simulink model "Elevator_simulation_regenerative_braking_completed"  (R2025b)
settings: Solver=VariableStepAuto  StartTime=0.0  StopTime=41  RelTol=1e-3
model workspace (MAT data in the model file):
  AFE_id_ref_profile = timeseries
  AFE_id_ref_profile.Name = 'unnamed'
  AFE_id_ref_profile.DataInfo = tsdata.datametadata
  AFE_id_ref_profile.DataInfo.Interpolation = tsdata.interpolation
  AFE_id_ref_profile.DataInfo.Interpolation.Fhandle : function handle (value not decoded)
  AFE_id_ref_profile.DataInfo.Interpolation.Name = 'linear'
  AFE_id_ref_profile.TimeInfo = tsdata.timemetadata
  AFE_id_ref_profile.TimeInfo.Length = 6
  AFE_id_ref_profile.TimeInfo.DuplicateTimes = 0
  AFE_id_ref_profile.TimeInfo.Time_ = [0; 0.1; 2; 3; 3.1; 5]
  AFE_id_ref_profile.TimeInfo.Initialized = 1
  AFE_id_ref_profile.QualityInfo = tsdata.qualmetadata
  AFE_id_ref_profile.Data_ = [0.5; 0.5; 0.5; 0.5; -0.5; -0.5]
  G = 10
  Jeq = 0.8325
  Tgravity = 27.25
  eta = 0.9
  g = 9.81
  mc = 500
  mcw = 600
  mp = 200
  r = 0.25
  regen_enable = timeseries
  regen_enable.Name = 'Regenerative braking enable'
  regen_enable.DataInfo = tsdata.datametadata
  regen_enable.DataInfo.Interpolation = tsdata.interpolation
  regen_enable.DataInfo.Interpolation.Fhandle : function handle (value not decoded)
  regen_enable.DataInfo.Interpolation.Name = 'linear'
  regen_enable.TimeInfo = tsdata.timemetadata
  regen_enable.TimeInfo.Length = 4
  regen_enable.TimeInfo.DuplicateTimes = 0
  regen_enable.TimeInfo.Time_ = [0; 0.2; 2.5; 5]
  regen_enable.TimeInfo.Initialized = 1
  regen_enable.QualityInfo = tsdata.qualmetadata
  regen_enable.Data_ = reshape([0 0 1 1], [1 1 4])
  sc_Pdead = 50
  sc_Plimit = 100000
  sc_Vinit = 360
  sc_Vmax = 470
  sc_Vmin = 300
  sc_dV = 10
  sc_enable = 1
  sc_kdis = 0.5
  sc_tauP = 0.02
  sc_tauV = 0.001
  speed_cmd = timeseries
  speed_cmd.Name = 'Elevator speed reference (round trip)'
  speed_cmd.DataInfo = tsdata.datametadata
  speed_cmd.DataInfo.Interpolation = tsdata.interpolation
  speed_cmd.DataInfo.Interpolation.Fhandle : function handle (value not decoded)
  speed_cmd.DataInfo.Interpolation.Name = 'linear'
  speed_cmd.TimeInfo = tsdata.timemetadata
  speed_cmd.TimeInfo.Length = 9
  speed_cmd.TimeInfo.DuplicateTimes = 0
  speed_cmd.TimeInfo.Time_ = [0; 8.001; 10.001; 18.001; 22; 30.001; 32.001; 40.001; 41]
  speed_cmd.TimeInfo.Initialized = 1
  speed_cmd.QualityInfo = tsdata.qualmetadata
  speed_cmd.Data_ = [0; 764; 764; 0; 0; -764; -764; 0; 0]
  speed_mps = timeseries
  speed_mps.Name = 'unnamed'
  speed_mps.DataInfo = tsdata.datametadata
  speed_mps.DataInfo.Interpolation = tsdata.interpolation
  speed_mps.DataInfo.Interpolation.Fhandle : function handle (value not decoded)
  speed_mps.DataInfo.Interpolation.Name = 'linear'
  speed_mps.TimeInfo = tsdata.timemetadata
  speed_mps.TimeInfo.Length = 4
  speed_mps.TimeInfo.DuplicateTimes = 0
  speed_mps.TimeInfo.Time_ = [0; 0.2; 2.5; 5]
  speed_mps.TimeInfo.Initialized = 1
  speed_mps.QualityInfo = tsdata.qualmetadata
  speed_mps.Data_ = [0; 2; 2; 0]
libraries: slpidlib x3, spsThreePhaseSeriesRLCBranchLib x3, spsThreePhaseVIMeasurementLib x3, spsControlledCurrentSourceLib x2, spsUniversalBridgeLib x2, spsVoltageMeasurementLib x2, autolibdcdc x1, spsCurrentMeasurementLib x1, eeGeneralControl x1, spsPLL3phLib x1, eePmsmFieldOrientedControl x1, spsPWMGenerator2LevelLib x1
settings Model: SimulationMode=rapid-accelerator  Creator=kesav  LastModifiedBy=kesava-d-raj
settings SolverCC: ZeroCrossAlgorithm=Adaptive

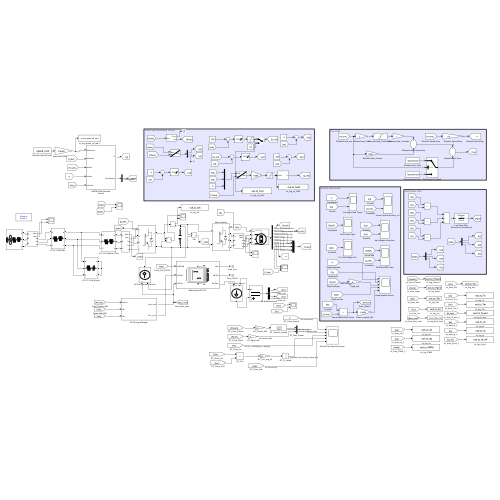
[thumbnail: Simulink's stored preview of the top-level diagram]
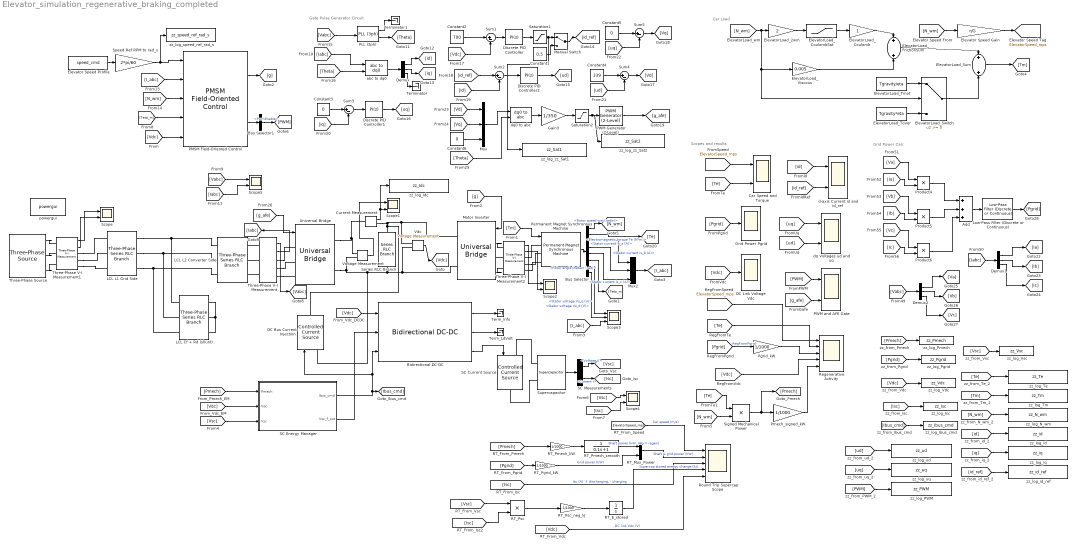
== system Elevator_simulation_regenerative_braking_completed ==
  note: Scopes and results
  note: Grid Power Calc
  note: Car Load
  note: Gate Pulse Generator Circuit
  Add : Sum  Inputs=+++
  Bidirectional DC-DC : autolibdcdc/Bidirectional DC-DC  Tc=1/1000  Vinit=0  Plimit=100000  param_loss=Single efficiency measurement  eff=98  v_loss_bp=[0 200 400 600 800 1000]  i_loss_bp=[0 25 50 75 100]  losses_table=[100 100 100 100 100;100 150 200 250 300;100 200 300 400 500;100 250 400 550 700;100 300 500 700 900;100 350 600 850 1100]  v_eff_bp=[200 400 600 800 1000]  i_eff_bp=[25 50 75 100]  efficiency_table=[96.2 98.1 98.7 99;98.1 99 99.4 99.5;98.7 99.4 99.6 99.7;99 99.5 99.7 99.8;99.2 99.6 99.7 99.8]  x_v_bp=[-1000 -800 -600 -400 -200 200 400 600 800 1000]  x_i_bp=[-100 -75 -50 -25 25 50 75 100]  x_losses_mat=[200.400801603196 225.67703109328 200.803212851408 201.612903225806 199.999999999997 200 225 200;160.320641282556 180.541624874624 201.005025125625 202.020202020203 200 200 180 160;180.541624874624 180.722891566267 181.086519114686 197.568389057748 194.999999999999 179.999999999997 180 180;201.005025125625 181.086519114686 202.020202020203 193.67991845056 190 200 179.999999999997 200;202.020202020203 197.568389057748 193.67991845056 197.505197505197 190 190 194.999999999999 200;200 194.999999999999 190 190 197.505197505197 193.67991845056 197.568389057748 202.020202020203;200 179.999999999997 200 190 193.67991845056 202.020202020203 181.086519114686 201.005025125625;180 180 179.999999999997 194.999999999999 197.568389057748 181.086519114686 180.722891566267 180.541624874624;160 180 200 200 202.020202020203 201.005025125625 180.541624874624 160.320641282556;200 225 200 199.999999999997 201.612903225806 200.803212851408 225.67703109328 200.400801603196]  RefBlkName='autolibdcdc/Bidirectional DC-DC'  CalLossMapData={'BaseCageProjectFileName','';'BaseMbcProjectFileName','';'TaskName','Calibrate Inverter Loss Map';'ChildTasks',{{'DataName','';'TaskName','Import Loss Data'},{'TaskName','Generate Response Models'},{'TaskName','Generate Calibration'},{'TaskName','Update Block Parameters'}}}
  Bus Selector : BusSelector  OutputSignals=Rotor speed wm (rad/s),Electromagnetic torque Te (N*m),Stator current is_a (A),Stator current is_b (A),Stator current is_c (A),Rotor angle thetam (rad),Stator voltage Vs_q (V),Stator voltage Vs_d (V)
  Bus Selector1 : BusSelector  OutputSignals=PwmEnable
  Car Speed and Torque : Scope  NumInputPorts=2
      settings: ActiveDisplayYMinimum=-2.5140849185806631  ActiveDisplayYMaximum=2.51411750297212
  Constant1 : Constant  Value=0.5
  Constant2 : Constant  Value=700
  Constant3 : Constant  Value=0
  Constant4 : Constant  Value=339
  Constant5 : Constant  Value=0
  Constant6 : Constant  Value=0
  Current Measurement : spsCurrentMeasurementLib/Current Measurement  PhasorSimulation=off  OutputType=Complex  PSBequivalent=0
  DC Bus Current Injection : spsControlledCurrentSourceLib/Controlled Current Source  Initialize=on  Source_Type=AC  Amplitude=0  Phase=0  Frequency=0  Measurements=None
  DC Link Voltage Vdc : Scope
      settings: ActiveDisplayYMinimum=572.34967767738488  ActiveDisplayYMaximum=718.84953066041635  DataLoggingVariableName=ScopeData2
  Demux : Demux  Outputs=3
  Demux1 : Demux  Outputs=3
  Demux2 : Demux  Outputs=3
  Discrete PID Controller : slpidlib/PID Controller  Controller=PI  Form=Parallel  TimeDomain=Discrete-time  UseExternalTs=off  SampleTime=1e-4  IntegratorMethod=Forward Euler  FilterMethod=Forward Euler  ControllerParametersSource=internal  P=0.5  I=15  UseKiTs=off  D=0  UseExternalDerivativeSource=off  N=100  UseFilter=on  TunerSelectOption=Transfer Function Based (PID Tuner App)  InitialConditionSource=internal  InitialConditionForIntegrator=0  InitialConditionForFilter=0  DifferentiatorICPrevScaledInput=0  ExternalReset=none  TrackingMode=off  Kt=1  LimitOutput=on  SatLimitsSource=internal  UpperSaturationLimit=20  LowerSaturationLimit=-20  LinearizeAsGain=off  AntiWindupMode=clamping  Kb=1  LimitIntegrator=off  UpperIntegratorSaturationLimit=inf  LowerIntegratorSaturationLimit=-inf  POutMin=[]  POutMax=[]  IOutMin=[]  IOutMax=[]  DOutMin=[]  DOutMax=[]  NOutMin=[]  NOutMax=[]  SumOutMin=[]  SumOutMax=[]  SaturationOutMin=[]  SaturationOutMax=[]  PParamMin=[]  PParamMax=[]  IParamMin=[]  IParamMax=[]  DParamMin=[]  DParamMax=[]  NParamMin=[]  NParamMax=[]  KbParamMin=[]  KbParamMax=[]  KtParamMin=[]  KtParamMax=[]  KbOutMin=[]  KbOutMax=[]  KtOutMin=[]  KtOutMax=[]  IntegratorOutMin=[]  IntegratorOutMax=[]  FilterOutMin=[]  FilterOutMax=[]  SumI1OutMin=[]  SumI1OutMax=[]  SumI2OutMin=[]  SumI2OutMax=[]  SumI3OutMin=[]  SumI3OutMax=[]  SumI4OutMin=[]  SumI4OutMax=[]  SumDOutMin=[]  SumDOutMax=[]  DifferentiatorOutMin=[]  DifferentiatorOutMax=[]  FilterDiffOutCoefMin=[]  FilterDiffOutCoefMax=[]  ReciprocalOutMin=[]  ReciprocalOutMax=[]  SumDenOutMin=[]  SumDenOutMax=[]  SumNumOutMin=[]  SumNumOutMax=[]  DivideOutMin=[]  DivideOutMax=[]  UdiffTsProdOutMin=[]  UdiffTsProdOutMax=[]  NTsProdOutMin=[]  NTsProdOutMax=[]  UintegralTsProdOutMin=[]  UintegralTsProdOutMax=[]  UngainTsProdOutMin=[]  UngainTsProdOutMax=[]  ClampingZeroOutDataTypeStr=Inherit: Inherit via back propagation  ClampingZeroOutMin=[]  ClampingZeroOutMax=[]  FilterDenConstantOutDataTypeStr=Inherit: Inherit via back propagation  FilterDenConstantOutMin=[]  FilterDenConstantOutMax=[]  PCopyOutDataTypeStr=Inherit: Inherit via back propagation  PCopyOutMin=[]  PCopyOutMax=[]  NCopyOutDataTypeStr=Inherit: Inherit via back propagation  NCopyOutMin=[]  NCopyOutMax=[]  IntegratorContinuousStateAttributes=''  IntegratorStateMustResolveToSignalObject=off  IntegratorRTWStateStorageClass=Auto  FilterContinuousStateAttributes=''  FilterStateMustResolveToSignalObject=off  FilterRTWStateStorageClass=Auto  ParallelPVariant=InternalParameters  IdealPVariant=Disabled  IVariant=InternalParameters  DVariant=Disabled  IntegratorVariant=Discrete  SatVariant=Enabled  AWVariant=DiscClampingParallel  PCopyVariant=Disabled  TRVariant=Disabled  FdbkBlocksVariant=Forward  IdealPFdbkVariant=Disabled  SatFdbkVariant=Disabled  DerivativeFilterVariant=Disabled  NVariant=Disabled  NCopyVariant=Disabled_SignalSpec  FilterICVariant=Disabled  IntegratorICVariant=InternalICs  ExternalResetVariant=Disabled  TRSumVariant=Passthrough  SumFdbkVariant=Disabled  SumVariant=Sum_PI  TsampFilterVariant=InternalTs  TsampNgainVariant=Passthrough  TsampIntegralVariant=Disabled_SignalSpec  ExternalSaturationOutDataTypeStr=Inherit: Same as second input  DerivativeSourceVariant=Disabled  PreIntVariant=InternalPreInt
      settings: LibrarySourceBlock=simulink/Discrete/Discrete PID Controller
  Discrete PID Controller1 : slpidlib/PID Controller  Controller=PI  Form=Parallel  TimeDomain=Discrete-time  UseExternalTs=off  SampleTime=5e-6  IntegratorMethod=Forward Euler  FilterMethod=Forward Euler  ControllerParametersSource=internal  P=15  I=30  UseKiTs=off  D=0  UseExternalDerivativeSource=off  N=100  UseFilter=on  TunerSelectOption=Transfer Function Based (PID Tuner App)  InitialConditionSource=internal  InitialConditionForIntegrator=0  InitialConditionForFilter=0  DifferentiatorICPrevScaledInput=0  ExternalReset=none  TrackingMode=off  Kt=1  LimitOutput=on  SatLimitsSource=internal  UpperSaturationLimit=350  LowerSaturationLimit=-350  LinearizeAsGain=off  AntiWindupMode=clamping  Kb=1  LimitIntegrator=off  UpperIntegratorSaturationLimit=inf  LowerIntegratorSaturationLimit=-inf  POutMin=[]  POutMax=[]  IOutMin=[]  IOutMax=[]  DOutMin=[]  DOutMax=[]  NOutMin=[]  NOutMax=[]  SumOutMin=[]  SumOutMax=[]  SaturationOutMin=[]  SaturationOutMax=[]  PParamMin=[]  PParamMax=[]  IParamMin=[]  IParamMax=[]  DParamMin=[]  DParamMax=[]  NParamMin=[]  NParamMax=[]  KbParamMin=[]  KbParamMax=[]  KtParamMin=[]  KtParamMax=[]  KbOutMin=[]  KbOutMax=[]  KtOutMin=[]  KtOutMax=[]  IntegratorOutMin=[]  IntegratorOutMax=[]  FilterOutMin=[]  FilterOutMax=[]  SumI1OutMin=[]  SumI1OutMax=[]  SumI2OutMin=[]  SumI2OutMax=[]  SumI3OutMin=[]  SumI3OutMax=[]  SumI4OutMin=[]  SumI4OutMax=[]  SumDOutMin=[]  SumDOutMax=[]  DifferentiatorOutMin=[]  DifferentiatorOutMax=[]  FilterDiffOutCoefMin=[]  FilterDiffOutCoefMax=[]  ReciprocalOutMin=[]  ReciprocalOutMax=[]  SumDenOutMin=[]  SumDenOutMax=[]  SumNumOutMin=[]  SumNumOutMax=[]  DivideOutMin=[]  DivideOutMax=[]  UdiffTsProdOutMin=[]  UdiffTsProdOutMax=[]  NTsProdOutMin=[]  NTsProdOutMax=[]  UintegralTsProdOutMin=[]  UintegralTsProdOutMax=[]  UngainTsProdOutMin=[]  UngainTsProdOutMax=[]  ClampingZeroOutDataTypeStr=Inherit: Inherit via back propagation  ClampingZeroOutMin=[]  ClampingZeroOutMax=[]  FilterDenConstantOutDataTypeStr=Inherit: Inherit via back propagation  FilterDenConstantOutMin=[]  FilterDenConstantOutMax=[]  PCopyOutDataTypeStr=Inherit: Inherit via back propagation  PCopyOutMin=[]  PCopyOutMax=[]  NCopyOutDataTypeStr=Inherit: Inherit via back propagation  NCopyOutMin=[]  NCopyOutMax=[]  IntegratorContinuousStateAttributes=''  IntegratorStateMustResolveToSignalObject=off  IntegratorRTWStateStorageClass=Auto  FilterContinuousStateAttributes=''  FilterStateMustResolveToSignalObject=off  FilterRTWStateStorageClass=Auto  ParallelPVariant=InternalParameters  IdealPVariant=Disabled  IVariant=InternalParameters  DVariant=Disabled  IntegratorVariant=Discrete  SatVariant=Enabled  AWVariant=DiscClampingParallel  PCopyVariant=Disabled  TRVariant=Disabled  FdbkBlocksVariant=Forward  IdealPFdbkVariant=Disabled  SatFdbkVariant=Disabled  DerivativeFilterVariant=Disabled  NVariant=Disabled  NCopyVariant=Disabled_SignalSpec  FilterICVariant=Disabled  IntegratorICVariant=InternalICs  ExternalResetVariant=Disabled  TRSumVariant=Passthrough  SumFdbkVariant=Disabled  SumVariant=Sum_PI  TsampFilterVariant=InternalTs  TsampNgainVariant=Passthrough  TsampIntegralVariant=Disabled_SignalSpec  ExternalSaturationOutDataTypeStr=Inherit: Same as second input  DerivativeSourceVariant=Disabled  PreIntVariant=InternalPreInt
      settings: LibrarySourceBlock=simulink/Discrete/Discrete PID Controller
  Discrete PID Controller2 : slpidlib/PID Controller  Controller=PI  Form=Parallel  TimeDomain=Discrete-time  UseExternalTs=off  SampleTime=5e-6  IntegratorMethod=Forward Euler  FilterMethod=Forward Euler  ControllerParametersSource=internal  P=15  I=30  UseKiTs=off  D=0  UseExternalDerivativeSource=off  N=100  UseFilter=on  TunerSelectOption=Transfer Function Based (PID Tuner App)  InitialConditionSource=internal  InitialConditionForIntegrator=0  InitialConditionForFilter=0  DifferentiatorICPrevScaledInput=0  ExternalReset=none  TrackingMode=off  Kt=1  LimitOutput=on  SatLimitsSource=internal  UpperSaturationLimit=350  LowerSaturationLimit=-350  LinearizeAsGain=off  AntiWindupMode=clamping  Kb=1  LimitIntegrator=off  UpperIntegratorSaturationLimit=inf  LowerIntegratorSaturationLimit=-inf  POutMin=[]  POutMax=[]  IOutMin=[]  IOutMax=[]  DOutMin=[]  DOutMax=[]  NOutMin=[]  NOutMax=[]  SumOutMin=[]  SumOutMax=[]  SaturationOutMin=[]  SaturationOutMax=[]  PParamMin=[]  PParamMax=[]  IParamMin=[]  IParamMax=[]  DParamMin=[]  DParamMax=[]  NParamMin=[]  NParamMax=[]  KbParamMin=[]  KbParamMax=[]  KtParamMin=[]  KtParamMax=[]  KbOutMin=[]  KbOutMax=[]  KtOutMin=[]  KtOutMax=[]  IntegratorOutMin=[]  IntegratorOutMax=[]  FilterOutMin=[]  FilterOutMax=[]  SumI1OutMin=[]  SumI1OutMax=[]  SumI2OutMin=[]  SumI2OutMax=[]  SumI3OutMin=[]  SumI3OutMax=[]  SumI4OutMin=[]  SumI4OutMax=[]  SumDOutMin=[]  SumDOutMax=[]  DifferentiatorOutMin=[]  DifferentiatorOutMax=[]  FilterDiffOutCoefMin=[]  FilterDiffOutCoefMax=[]  ReciprocalOutMin=[]  ReciprocalOutMax=[]  SumDenOutMin=[]  SumDenOutMax=[]  SumNumOutMin=[]  SumNumOutMax=[]  DivideOutMin=[]  DivideOutMax=[]  UdiffTsProdOutMin=[]  UdiffTsProdOutMax=[]  NTsProdOutMin=[]  NTsProdOutMax=[]  UintegralTsProdOutMin=[]  UintegralTsProdOutMax=[]  UngainTsProdOutMin=[]  UngainTsProdOutMax=[]  ClampingZeroOutDataTypeStr=Inherit: Inherit via back propagation  ClampingZeroOutMin=[]  ClampingZeroOutMax=[]  FilterDenConstantOutDataTypeStr=Inherit: Inherit via back propagation  FilterDenConstantOutMin=[]  FilterDenConstantOutMax=[]  PCopyOutDataTypeStr=Inherit: Inherit via back propagation  PCopyOutMin=[]  PCopyOutMax=[]  NCopyOutDataTypeStr=Inherit: Inherit via back propagation  NCopyOutMin=[]  NCopyOutMax=[]  IntegratorContinuousStateAttributes=''  IntegratorStateMustResolveToSignalObject=off  IntegratorRTWStateStorageClass=Auto  FilterContinuousStateAttributes=''  FilterStateMustResolveToSignalObject=off  FilterRTWStateStorageClass=Auto  ParallelPVariant=InternalParameters  IdealPVariant=Disabled  IVariant=InternalParameters  DVariant=Disabled  IntegratorVariant=Discrete  SatVariant=Enabled  AWVariant=DiscClampingParallel  PCopyVariant=Disabled  TRVariant=Disabled  FdbkBlocksVariant=Forward  IdealPFdbkVariant=Disabled  SatFdbkVariant=Disabled  DerivativeFilterVariant=Disabled  NVariant=Disabled  NCopyVariant=Disabled_SignalSpec  FilterICVariant=Disabled  IntegratorICVariant=InternalICs  ExternalResetVariant=Disabled  TRSumVariant=Passthrough  SumFdbkVariant=Disabled  SumVariant=Sum_PI  TsampFilterVariant=InternalTs  TsampNgainVariant=Passthrough  TsampIntegralVariant=Disabled_SignalSpec  ExternalSaturationOutDataTypeStr=Inherit: Same as second input  DerivativeSourceVariant=Disabled  PreIntVariant=InternalPreInt
      settings: LibrarySourceBlock=simulink/Discrete/Discrete PID Controller
  Elevator Speed Gain : Gain  Gain=r/G
  Elevator Speed Profile : FromWorkspace  VariableName=speed_cmd  OutputAfterFinalValue=Holding final value
  ElevatorLoad_2wm : Gain  Gain=2
  ElevatorLoad_Coulomb : Gain
  ElevatorLoad_CoulombSat : Saturate  UpperLimit=1  LowerLimit=-1
  ElevatorLoad_FrictionSum : Sum
  ElevatorLoad_Sum : Sum
  ElevatorLoad_Switch : Switch  SaturateOnIntegerOverflow=off  InputSameDT=off
  ElevatorLoad_Tmot : Constant  Value=Tgravity/eta
  ElevatorLoad_Tover : Constant  Value=Tgravity*eta
  ElevatorLoad_Viscous : Gain  Gain=0.005
  Gain3 : Gain  Gain=1/350
  Grid Power Pgrid : Scope
      settings: ActiveDisplayYMinimum=-251.99323662380996  ActiveDisplayYMaximum=2303.7936894253148  DataLoggingVariableName=ScopeData3
  LCL Cf + Rd (shunt) : spsThreePhaseSeriesRLCBranchLib/Three-Phase Series RLC Branch  LConnTagsString=A|B|C  RConnTagsString=A|B|C  BranchType=RC  Resistance=3.93178  Inductance=1e-3  Capacitance=9.24111e-06  Measurements=None
  LCL L1 Grid Side : spsThreePhaseSeriesRLCBranchLib/Three-Phase Series RLC Branch  LConnTagsString=A|B|C  RConnTagsString=A|B|C  BranchType=RL  Resistance=0.01  Inductance=0.0013  Capacitance=1e-6  Measurements=None
  LCL L2 Converter Side : spsThreePhaseSeriesRLCBranchLib/Three-Phase Series RLC Branch  LConnTagsString=A|B|C  RConnTagsString=A|B|C  BranchType=RL  Resistance=0.03  Inductance=0.0045  Capacitance=1e-6  Measurements=None
  Low-Pass Filter (Discrete or Continuous) : eeGeneralControl/Low-Pass Filter (Discrete or Continuous)  K=1  T=0.1  B=inf  A=-inf  init_option=Inherited from block input  x0=0  Ts=-1
  Manual Switch : ManualSwitch
  Motor Inverter : spsUniversalBridgeLib/Universal Bridge  Arms=3  SnubberResistance=1e5  SnubberCapacitance=inf  Device=IGBT / Diodes  Ron=1e-3  Lon=0  ForwardVoltages="[  0  0  ]"  ForwardVoltage=0  GTOparameters=[ 10e-6 , 20e-6 ]  IGBTparameters=[ 1e-6 , 2e-6 ]  Measurements=None  Measurements_2=None  converterType=Rectifier
  Mux : Mux  Inputs=3
  Mux2 : Mux  Inputs=3
  PLL (3ph) : spsPLL3phLib/PLL (3ph)  Fmin=45  Par_Init=[0, 50]  ParK=[180, 3200, 1]  TcD=1e-4  MaxRateChangeFreq=12  FilterCutOffFreq=25  Ts=1e-4  AGC=on
  PMSM Field-Oriented Control : eePmsmFieldOrientedControl/PMSM Field-Oriented Control  winding_type=Wye-wound  CtrlMode=Velocity control  Vnom=560  Pmax=75000  Tmax=40  p=4  Vdc_on=100  Ts=5e-6  Tsc=1e-4  CtrlType=PI control  Kp_w=15  Ki_w=50  Kv_w=1  Kaw_w=10  RefType=Zero d-axis control  rpmVec=[0, 3000]  TqVec=[-100, 0, 100]  VdcVec=[300, 350]  PWMMode=SVM: space vector modulation  ModFactor=1  idMatrix=zeros(2,3,2)  iqMatrix=zeros(2,3,2)  psim=0.1194  Ld=0.0085  Lq=0.0085  Rs=0.5  AxisAlignment=D-axis  Kp_id=0.745  Ki_id=91  Kaw_id=1  Kp_iq=0.745  Ki_iq=91  Kaw_iq=1  AxisPrio=Q-axis  ActZC=off  ActFF=on  ParamTypeFF=Constant parameters  LdFF=0.0085  LqFF=0.0085  psimFF=0.1194  idVect=[-200, 0, 200]  iqVect=[-200, 0, 200]  LdMatrix=0.0002 * ones(3, 3)  LqMatrix=0.0002 * ones(3, 3)  psimMatrix=0.04 * ones(3, 3)  CPWMMode=SVM: space vector modulation  fsw=1000
      settings: LibrarySourceBlock=|
      | ee_sl_lib/PMSM Control/PMSM Field-Oriented
      | Control
  PWM Generator (2-Level) : spsPWMGenerator2LevelLib/PWM Generator (2-Level)  ModulatorType=Three-phase bridge (6 pulses)  ModulatorMode=Unsynchronized  Fc=5000  Pc=90  nF=27  MinMax="[ -1  1 ]"  SamplingTechnique=Natural  ModulatingSignals=off  m=0.8  Freq=60  Phase=0  Ts=0  ShowCarrierOutport=off
  PWM and AFE Gate : Scope  NumInputPorts=2
      settings: ActiveDisplayYMinimum=-1  ActiveDisplayYMaximum=1  DataLoggingVariableName=ScopeData4
  Permanent Magnet Synchronous Machine : spsPermanentMagnetSynchronousMachineLib/Permanent Magnet Synchronous Machine  NbPhases=3  FluxDistribution=Sinusoidal  RotorType=Round  MechanicalLoad=Torque Tm  PresetModel=No  ShowDetailedParameters=on  MeasurementBus=off  Resistance=0.5  Inductance=8.5e-3  dqInductances=[8.5e-3,8.5e-3]  La=7e-3  MachineConstant=Flux linkage established by magnets (V.s)  Flux=0.1194  VoltageCst=86.6271  TorqueCst=0.7164  Flat=120  Mechanical=[Jeq 0.0004924 4 0]  PolePairs=4  InitialConditions=[0,0, 0,0]  InitialConditions5ph=[0 0 0 0 0 0]  RefAngle=Aligned with phase A axis (original Park)  IterativeDiscreteModel=Trapezoidal non iterative  TsBlock=-1  TsPowergui=0
  Pgrid_kW : Gain  Gain=1/1000
  Pmech_signed_kW : Gain  Gain=1/1000
  Product4 : Product
  Product5 : Product
  Product6 : Product
  RT_E_stored : Integrator
  RT_Mux_Power : Mux  Inputs=2
  RT_Pgrid_kW : Gain  Gain=1/1000
  RT_Pmech_kW : Gain  Gain=1/1000
  RT_Pmech_smooth : TransferFcn  Denominator=[0.1 1]
  RT_Psc : Product  Inputs=**
  RT_Psc_neg_kJ : Gain  Gain=-1/1000
  Regenerative Activity : Scope  NumInputPorts=5
      settings: ActiveDisplayYMinimum=-2.5140849185806631  ActiveDisplayYMaximum=2.51411750297212  DataLoggingVariableName=regenScopeData
  Round Trip Supercap Scope : Scope  NumInputPorts=5
      settings: Title=Round trip: up, door pause, down  DataLoggingVariableName=zz_scope_rt
  SC Current Source : spsControlledCurrentSourceLib/Controlled Current Source  Initialize=on  Source_Type=AC  Amplitude=0  Phase=0  Frequency=0  Measurements=None
  SC Energy Manager : Subsystem
  SC Measurements : BusSelector  OutputSignals=Voltage V,Current I
  Saturation1 : Saturate  UpperLimit=20  LowerLimit=-20
  Saturation2 : Saturate  UpperLimit=1  LowerLimit=-1
  Scope{,1..2,4..5} (5 alike) : Scope  NumInputPorts=2
      Scope settings: ActiveDisplayYMinimum=-427.79945826424978  ActiveDisplayYMaximum=427.95539534546936  DataLoggingVariableName=ScopeData6
      Scope1 settings: ActiveDisplayYMinimum=572.34967767738488  ActiveDisplayYMaximum=718.84953066041635  DataLoggingVariableName=ScopeData7
      Scope2 settings: ActiveDisplayYMinimum=-875.88810158987451  ActiveDisplayYMaximum=875.79768155604654  DataLoggingVariableName=ScopeData8
      Scope4 settings: ActiveDisplayYMinimum=260  ActiveDisplayYMaximum=460  DataLoggingVariableName=ScopeData10
      Scope5 settings: ActiveDisplayYMinimum=-583.8618425867395  ActiveDisplayYMaximum=583.86292243007767  DataLoggingVariableName=ScopeData11
  Scope3 : Scope  NumInputPorts=3
      settings: ActiveDisplayYMinimum=-451.32528347308204  ActiveDisplayYMaximum=569.01573785886433  DataLoggingVariableName=ScopeData9
  Series RLC Branch : spsSeriesRLCBranchLib/Series RLC Branch  LConnTagsString=__new0  RConnTagsString=__new0  BranchType=C  Resistance=0.01  Inductance=1e-3  SetiL0=off  InitialCurrent=0  Capacitance=3e-3  Setx0=on  InitialVoltage=587  Measurements=None
  Signed Mechanical Power : Product  Inputs=**
  Speed Ref RPM to rad_s : Gain  Gain=2*pi/60
  Sum{1..5} (5 alike) : Sum  Inputs=|+-
  Supercapacitor : spsSupercapacitorLib/Supercapacitor  C=99.5  Rdc=8.9e-3  Voltage=48  Ns=10  Np=1  Vinit=sc_Vinit  Temp=25  Nc=1  r=1e-9  epsilon=6.0208e-10  Ioc=10  Vself="[48  47.8  47.06  44.65]"
      settings: LibrarySourceBlock=sps_lib/Sources/Supercapacitor
  Term_Info : Terminator
  Term_LdVolt : Terminator
  Terminator : Terminator
  Terminator1 : Terminator
  Three-Phase V-I Measurement : spsThreePhaseVIMeasurementLib/Three-Phase V-I Measurement  VoltageMeasurement=phase-to-ground  SetLabelV=off  LabelV=Vabc  Vpu=off  VpuLL=off  CurrentMeasurement=yes  SetLabelI=off  LabelI=Iabc  Ipu=off  Pbase=100e6  Vbase=500e3  OutputType=Complex  PhasorSimulation=off  PSBequivalent=0
  Three-Phase V-I Measurement1 : spsThreePhaseVIMeasurementLib/Three-Phase V-I Measurement  VoltageMeasurement=phase-to-ground  SetLabelV=off  LabelV=Vabc  Vpu=off  VpuLL=off  CurrentMeasurement=yes  SetLabelI=off  LabelI=Iabc  Ipu=off  Pbase=100e6  Vbase=500e3  OutputType=Complex  PhasorSimulation=off  PSBequivalent=0
  Three-Phase V-I Measurement2 : spsThreePhaseVIMeasurementLib/Three-Phase V-I Measurement  VoltageMeasurement=phase-to-ground  SetLabelV=off  LabelV=Vabc  Vpu=off  VpuLL=off  CurrentMeasurement=yes  SetLabelI=off  LabelI=Iabc  Ipu=off  Pbase=100e6  Vbase=500e3  OutputType=Complex  PhasorSimulation=off  PSBequivalent=0
  Three-Phase Source : spsThreePhaseSourceLib/Three-Phase Source  InternalConnection=Yg  VoltagePhases=off  Voltage=415  PhaseAngle=0  Voltage_phases=[25e3 25e3 25e3]/sqrt(3)  PhaseAngles_phases=[0 -120 +120]  Frequency=50  NonIdealSource=on  SpecifyImpedance=off  Resistance=0.05  Inductance=0.5e-3  ShortCircuitLevel=100e6  BaseVoltage=25e3  XRratio=7  BusType=swing  Pref=10e3  Qref=0  Prefabc=[10e3, 10e3, 10e3]  Qrefabc=[0, 0, 0]  Qmin=-inf  Qmax=inf
  Universal Bridge : spsUniversalBridgeLib/Universal Bridge  Arms=3  SnubberResistance=1e5  SnubberCapacitance=inf  Device=IGBT / Diodes  Ron=1e-3  Lon=0  ForwardVoltages="[  0  0  ]"  ForwardVoltage=0  GTOparameters=[ 10e-6 , 20e-6 ]  IGBTparameters=[ 1e-6 , 2e-6 ]  Measurements=None  Measurements_2=None  converterType=Rectifier
  Vdc : spsVoltageMeasurementLib/Voltage Measurement  PhasorSimulation=off  OutputType=Complex  PSBequivalent=0
  Voltage Measurement : spsVoltageMeasurementLib/Voltage Measurement  PhasorSimulation=off  OutputType=Complex  PSBequivalent=0
  abc to dq0 : spsabctodq0Lib/abc to dq0  Alignment=90 degrees behind phase A axis
  d-axis Current id and id_ref : Scope  NumInputPorts=2
      settings: ActiveDisplayYMinimum=-6.2747830010802819  ActiveDisplayYMaximum=32.204392109393645  DataLoggingVariableName=ScopeData5
  dq Voltages ud and uq : Scope  NumInputPorts=2
      settings: ActiveDisplayYMinimum=-197.76555439182147  ActiveDisplayYMaximum=355.20674335903738
  dq0 to abc : spsdq0toabcLib/dq0 to abc  Alignment=90 degrees behind phase A axis
  powergui : sps_lib/powergui  Priority=1  SimulationMode=Discrete  SampleTime=5e-6  frequency=60  Iterations=50  frequencyindice=0  Pbase=100e6  ErrMax=1e-4  UnitsV=kV  UnitsW=MW  buscounter=0  FunctionMessages=off  echomessages=off  EnableUseOfTLC=off  CurrentSourceSwitches=off  DisableSnubberDevices=off  DisableRonSwitches=off  DisableVfSwitches=off  DisplayEquations=off  AutomaticDiscreteSolvers=off  SolverType=Tustin/Backward Euler (TBE)  Interpol=off  ExternalGateDelay=off  methode=off  Ts=100  x0status=blocks  SPID=on  SwTol=0  HookPort=off  NonlinearTolerance=1e-4  nMaxIteration=100  ContinueOnMaxIteration=off  RestoreLinks=warning  ResistiveCurrentMeasurement=off  Frange=[0:2:500]  Ylog=off  Xlog=on  ShowGrid=off  save=off  variable=ZData  structure=0  ZoomFFT=off  StartTime=0.0  cycles=1  DisplayStyle=1  fundamental=60  FreqAxis=off  MaxFrequency=1000  frequencyindicesteady=1  RmsSteady=1  display=off
  zz_log_Ibus_cmd : ToWorkspace  VariableName=zz_Ibus_cmd  SaveFormat=Timeseries  SampleTime=1e-3
  zz_log_Idc : ToWorkspace  VariableName=zz_Idc  SaveFormat=Timeseries  SampleTime=1e-3
  zz_log_Isc : ToWorkspace  VariableName=zz_Isc  SaveFormat=Timeseries  SampleTime=1e-3
  zz_log_N_wm : ToWorkspace  VariableName=zz_N_wm  SaveFormat=Timeseries  SampleTime=1e-3
  zz_log_PWM : ToWorkspace  VariableName=zz_PWM  SaveFormat=Timeseries  SampleTime=1e-3
  zz_log_Pgrid : ToWorkspace  VariableName=zz_Pgrid  SaveFormat=Timeseries  SampleTime=1e-3
  zz_log_Pmech : ToWorkspace  VariableName=zz_Pmech  SaveFormat=Timeseries  SampleTime=1e-3
  zz_log_Te : ToWorkspace  VariableName=zz_Te  SaveFormat=Timeseries  SampleTime=1e-3
  zz_log_Tm : ToWorkspace  VariableName=zz_Tm  SaveFormat=Timeseries  SampleTime=1e-3
  zz_log_Vdc : ToWorkspace  VariableName=zz_Vdc  SaveFormat=Timeseries  SampleTime=1e-3
  zz_log_Vsc : ToWorkspace  VariableName=zz_Vsc  SaveFormat=Timeseries  SampleTime=1e-3
  zz_log_id : ToWorkspace  VariableName=zz_id  SaveFormat=Timeseries  SampleTime=1e-3
  zz_log_id_ref : ToWorkspace  VariableName=zz_id_ref  SaveFormat=Timeseries  SampleTime=1e-3
  zz_log_iq : ToWorkspace  VariableName=zz_iq  SaveFormat=Timeseries  SampleTime=1e-3
  zz_log_speed_ref_rad_s : ToWorkspace  VariableName=zz_speed_ref_rad_s  SaveFormat=Timeseries  SampleTime=-1
  zz_log_ud : ToWorkspace  VariableName=zz_ud  SaveFormat=Timeseries  SampleTime=1e-3
  zz_log_uq : ToWorkspace  VariableName=zz_uq  SaveFormat=Timeseries  SampleTime=1e-3
  zz_log_zz_Sat1 : ToWorkspace  VariableName=zz_Sat1  SaveFormat=Timeseries  SampleTime=1e-3
  zz_log_zz_Sat2 : ToWorkspace  VariableName=zz_Sat2  SaveFormat=Timeseries  SampleTime=1e-3
  tag scope: ElevatorSpeed_mps=global
  wires:
  Vdc/1 -> [Vdc]
  Permanent Magnet Synchronous Machine/1 -> Bus Selector/1
  [g] -> Motor Inverter/1
  Bus Selector/6 -> [Teta_m]  "<Rotor angle thetam (rad)>"
  Bus Selector/3 -> Mux2/1  "<Stator current is_a (A)>"
  Mux2/1 -> [I_abc]
  Bus Selector/4 -> Mux2/2  "<Stator current is_b (A)>"
  Bus Selector/5 -> Mux2/3  "<Stator current is_c (A)>"
  Bus Selector/1 -> [N_wm]  "<Rotor speed wm (rad/s)>"
  [I_abc] -> PMSM Field-Oriented Control/2
  [N_wm] -> PMSM Field-Oriented Control/3
  [Vdc] -> PMSM Field-Oriented Control/5
  PMSM Field-Oriented Control/2 -> Bus Selector1/1
  PMSM Field-Oriented Control/1 -> [g]
  Bus Selector1/1 -> [PWM]  "<PwmEnable>"
  [Teta_m] -> PMSM Field-Oriented Control/4
  Three-Phase V-I Measurement/1 -> [Vabc]
  Three-Phase V-I Measurement/2 -> [Iabc]
  [Vabc] -> PLL (3ph)/1
  PLL (3ph)/2 -> [Theta]
  [Theta] -> abc to dq0/2
  [Iabc] -> abc to dq0/1
  abc to dq0/1 -> Demux/1
  Demux/1 -> [id]
  Demux/2 -> [iq]
  Constant2/1 -> Sum1/1
  [Vdc] -> Sum1/2
  Sum1/1 -> Discrete PID Controller/1
  Discrete PID Controller/1 -> Saturation1/1
  [id_ref] -> Sum2/1
  [id] -> Sum2/2
  Sum2/1 -> Discrete PID Controller2/1
  Discrete PID Controller2/1 -> [ud]
  Sum3/1 -> Discrete PID Controller1/1
  Discrete PID Controller1/1 -> [uq]
  [iq] -> Sum3/2
  Constant3/1 -> Sum3/1
  PLL (3ph)/1 -> Terminator1/1
  Demux/3 -> Terminator/1
  Constant4/1 -> Sum4/1
  [ud] -> Sum4/2
  Sum4/1 -> [Vd]
  Sum5/1 -> [Vq]
  [uq] -> Sum5/2
  Constant5/1 -> Sum5/1
  [Vd] -> Mux/1
  [Vq] -> Mux/2
  Constant6/1 -> Mux/3
  Mux/1 -> dq0 to abc/1
  [Theta] -> dq0 to abc/2
  dq0 to abc/1 -> Gain3/1
  Gain3/1 -> Saturation2/1
  Saturation2/1 -> PWM Generator (2-Level)/1, zz_log_zz_Sat2/1
  PWM Generator (2-Level)/1 -> [g_afe]
  [g_afe] -> Universal Bridge/1
  Bus Selector/2 -> [Te]  "<Electromagnetic torque Te (N*m)>"
  [Iabc] -> Demux1/1
  Demux1/1 -> [Ia]
  Demux1/2 -> [Ib]
  Demux1/3 -> [Ic]
  Demux2/1 -> [Va]
  Demux2/3 -> [Vc]
  Demux2/2 -> [Vb]
  [Vabc] -> Demux2/1
  [Va] -> Product4/1
  [Ia] -> Product4/2
  [Ib] -> Product5/2
  [Vb] -> Product5/1
  [Ic] -> Product6/2
  [Vc] -> Product6/1
  Product4/1 -> Add/1
  Product5/1 -> Add/2
  Product6/1 -> Add/3
  Add/1 -> Low-Pass Filter (Discrete or Continuous)/1
  Low-Pass Filter (Discrete or Continuous)/1 -> [Pgrid]
  Saturation1/1 -> Manual Switch/1, zz_log_zz_Sat1/1
  Constant1/1 -> Manual Switch/2
  [N_wm] -> Elevator Speed Gain/1
  Elevator Speed Gain/1 -> [ElevatorSpeed_mps]
  [g_afe] -> PWM and AFE Gate/2
  [PWM] -> PWM and AFE Gate/1
  [ud] -> dq Voltages ud and uq/2
  [uq] -> dq Voltages ud and uq/1
  [Pgrid] -> Grid Power Pgrid/1
  [id] -> d-axis Current id and id_ref/1
  [id_ref] -> d-axis Current id and id_ref/2
  [Vdc] -> DC Link Voltage Vdc/1
  [ElevatorSpeed_mps] -> Regenerative Activity/1
  [Te] -> Regenerative Activity/2
  [Pgrid] -> Pgrid_kW/1  "RegFromPgrid"
  [Vdc] -> Regenerative Activity/4
  Pgrid_kW/1 -> Regenerative Activity/3
  [N_wm] -> ElevatorLoad_Viscous/1, ElevatorLoad_Switch/2, ElevatorLoad_2wm/1
  ElevatorLoad_2wm/1 -> ElevatorLoad_CoulombSat/1
  ElevatorLoad_CoulombSat/1 -> ElevatorLoad_Coulomb/1
  ElevatorLoad_Coulomb/1 -> ElevatorLoad_FrictionSum/1
  ElevatorLoad_Viscous/1 -> ElevatorLoad_FrictionSum/2
  ElevatorLoad_Tmot/1 -> ElevatorLoad_Switch/1
  ElevatorLoad_Tover/1 -> ElevatorLoad_Switch/3
  [Tm] -> Permanent Magnet Synchronous Machine/1
  ElevatorLoad_Sum/1 -> [Tm]
  ElevatorLoad_FrictionSum/1 -> ElevatorLoad_Sum/1
  ElevatorLoad_Switch/1 -> ElevatorLoad_Sum/2
  [ElevatorSpeed_mps] -> Car Speed and Torque/1
  [Te] -> Car Speed and Torque/2
  Manual Switch/1 -> [id_ref]
  Signed Mechanical Power/1 -> Pmech_signed_kW/1, [Pmech]
  Pmech_signed_kW/1 -> Regenerative Activity/5
  Three-Phase V-I Measurement1/1 -> Scope/1
  Three-Phase V-I Measurement1/2 -> Scope/2
  Current Measurement/1 -> Scope1/2, zz_log_Idc/1
  Voltage Measurement/1 -> Scope1/1
  Three-Phase V-I Measurement2/1 -> Scope2/1
  Three-Phase V-I Measurement2/2 -> Scope2/2
  Bus Selector/7 -> Scope3/1  "<Stator voltage Vs_q (V)>"
  Bus Selector/8 -> Scope3/2  "<Stator voltage Vs_d (V)>"
  [I_abc] -> Scope3/3
  Supercapacitor/1 -> SC Measurements/1
  [Pmech] -> SC Energy Manager/1(Pmech)
  [Vdc] -> SC Energy Manager/2(Vdc)
  SC Measurements/1 -> [Vsc]  "<Voltage V>"
  [Vdc] -> Bidirectional DC-DC/1
  SC Energy Manager/2(Vsc_f_out) -> Bidirectional DC-DC/2
  SC Energy Manager/1(Ibus_cmd) -> Bidirectional DC-DC/3, DC Bus Current Injection/1, [Ibus_cmd]
  Bidirectional DC-DC/1 -> Term_Info/1
  Bidirectional DC-DC/2 -> Term_LdVolt/1
  Bidirectional DC-DC/3 -> SC Current Source/1
  SC Measurements/2 -> [Isc]  "<Current I>"
  [Vsc] -> SC Energy Manager/3(Vsc)
  [Te] -> Signed Mechanical Power/1
  [N_wm] -> Signed Mechanical Power/2
  [Pmech] -> zz_log_Pmech/1
  [Pgrid] -> zz_log_Pgrid/1
  [Vdc] -> zz_log_Vdc/1
  [Vsc] -> zz_log_Vsc/1
  [Isc] -> zz_log_Isc/1
  [Ibus_cmd] -> zz_log_Ibus_cmd/1
  [Vsc] -> Scope4/1
  [Isc] -> Scope4/2
  [Te] -> zz_log_Te/1
  [Tm] -> zz_log_Tm/1
  [N_wm] -> zz_log_N_wm/1
  [id] -> zz_log_id/1
  [iq] -> zz_log_iq/1
  [id_ref] -> zz_log_id_ref/1
  [ud] -> zz_log_ud/1
  [uq] -> zz_log_uq/1
  [PWM] -> zz_log_PWM/1
  Elevator Speed Profile/1 -> Speed Ref RPM to rad_s/1
  Speed Ref RPM to rad_s/1 -> zz_log_speed_ref_rad_s/1, PMSM Field-Oriented Control/1
  [Vabc] -> Scope5/1
  [Iabc] -> Scope5/2
  [ElevatorSpeed_mps] -> Round Trip Supercap Scope/1  "Car speed (m/s)"
  [Pmech] -> RT_Pmech_kW/1
  RT_Pmech_kW/1 -> RT_Pmech_smooth/1
  RT_Pmech_smooth/1 -> RT_Mux_Power/1  "Shaft power (kW, neg = regen)"
  [Pgrid] -> RT_Pgrid_kW/1
  RT_Pgrid_kW/1 -> RT_Mux_Power/2  "Grid power (kW)"
  RT_Mux_Power/1 -> Round Trip Supercap Scope/2  "Shaft & grid power (kW)"
  [Isc] -> Round Trip Supercap Scope/3  "Isc (A): + discharging, - charging"
  [Vsc] -> RT_Psc/1
  [Isc] -> RT_Psc/2
  RT_Psc/1 -> RT_Psc_neg_kJ/1
  RT_Psc_neg_kJ/1 -> RT_E_stored/1
  RT_E_stored/1 -> Round Trip Supercap Scope/4  "Supercap stored energy change (kJ)"
  [Vdc] -> Round Trip Supercap Scope/5  "DC link Vdc (V)"
  connections:
  Three-Phase V-I Measurement/RConn3 -- Universal Bridge/LConn3
  Three-Phase V-I Measurement/RConn2 -- Universal Bridge/LConn2
  Three-Phase V-I Measurement/RConn1 -- Universal Bridge/LConn1
  Vdc/LConn2 -- Motor Inverter/RConn2 -- Voltage Measurement/LConn2 -- Universal Bridge/RConn2 -- DC Bus Current Injection/LConn1 -- Series RLC Branch/RConn1
  Universal Bridge/RConn1 -- Current Measurement/LConn1 -- Voltage Measurement/LConn1
  Three-Phase Source/RConn1 -- Three-Phase V-I Measurement1/LConn1
  Three-Phase Source/RConn2 -- Three-Phase V-I Measurement1/LConn2
  Three-Phase Source/RConn3 -- Three-Phase V-I Measurement1/LConn3
  Three-Phase V-I Measurement1/RConn1 -- LCL L1 Grid Side/LConn1
  Vdc/LConn1 -- Current Measurement/RConn1 -- Series RLC Branch/LConn1 -- DC Bus Current Injection/RConn1 -- Motor Inverter/RConn1
  Three-Phase V-I Measurement2/LConn2 -- Motor Inverter/LConn2
  Motor Inverter/LConn1 -- Three-Phase V-I Measurement2/LConn1
  Motor Inverter/LConn3 -- Three-Phase V-I Measurement2/LConn3
  Three-Phase V-I Measurement2/RConn1 -- Permanent Magnet Synchronous Machine/LConn1
  Three-Phase V-I Measurement2/RConn2 -- Permanent Magnet Synchronous Machine/LConn2
  Three-Phase V-I Measurement2/RConn3 -- Permanent Magnet Synchronous Machine/LConn3
  Supercapacitor/LConn1 -- SC Current Source/LConn1
  Supercapacitor/LConn2 -- SC Current Source/RConn1
  Three-Phase V-I Measurement1/RConn2 -- LCL L1 Grid Side/LConn2
  Three-Phase V-I Measurement1/RConn3 -- LCL L1 Grid Side/LConn3
  Three-Phase V-I Measurement/LConn1 -- LCL L2 Converter Side/RConn1
  Three-Phase V-I Measurement/LConn2 -- LCL L2 Converter Side/RConn2
  Three-Phase V-I Measurement/LConn3 -- LCL L2 Converter Side/RConn3
  LCL L1 Grid Side/RConn1 -- LCL Cf + Rd (shunt)/LConn1 -- LCL L2 Converter Side/LConn1
  LCL L1 Grid Side/RConn2 -- LCL L2 Converter Side/LConn2 -- LCL Cf + Rd (shunt)/LConn2
  LCL L1 Grid Side/RConn3 -- LCL L2 Converter Side/LConn3 -- LCL Cf + Rd (shunt)/LConn3
  LCL Cf + Rd (shunt)/RConn2 -- LCL Cf + Rd (shunt)/RConn1 -- LCL Cf + Rd (shunt)/RConn3

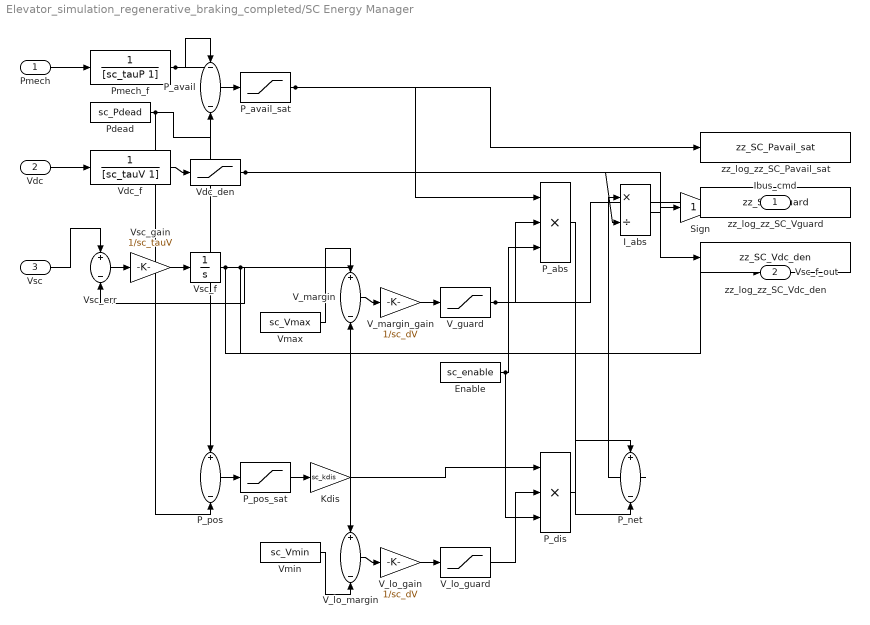
== system Elevator_simulation_regenerative_braking_completed/SC Energy Manager ==
  Pmech : Inport
  Vdc : Inport  Port=2
  Vsc : Inport  Port=3
  Enable : Constant  Value=sc_enable
  I_abs : Product  Inputs=*/
  Kdis : Gain  Gain=sc_kdis
  P_abs : Product  Inputs=***
  P_avail : Sum  Inputs=--
  P_avail_sat : Saturate  UpperLimit=sc_Plimit  LowerLimit=0
  P_dis : Product  Inputs=***
  P_net : Sum  Inputs=+-
  P_pos : Sum  Inputs=+-
  P_pos_sat : Saturate  UpperLimit=sc_Plimit  LowerLimit=0
  Pdead : Constant  Value=sc_Pdead
  Pmech_f : TransferFcn  Denominator=[sc_tauP 1]
  Sign : Gain
  V_guard : Saturate  UpperLimit=1  LowerLimit=0
  V_lo_gain : Gain  Gain=1/sc_dV
  V_lo_guard : Saturate  UpperLimit=1  LowerLimit=0
  V_lo_margin : Sum  Inputs=+-
  V_margin : Sum  Inputs=+-
  V_margin_gain : Gain  Gain=1/sc_dV
  Vdc_den : Saturate  UpperLimit=2000  LowerLimit=100
  Vdc_f : TransferFcn  Denominator=[sc_tauV 1]
  Vmax : Constant  Value=sc_Vmax
  Vmin : Constant  Value=sc_Vmin
  Vsc_err : Sum  Inputs=+-
  Vsc_f : Integrator  InitialCondition=sc_Vinit
  Vsc_gain : Gain  Gain=1/sc_tauV
  zz_log_zz_SC_Pavail_sat : ToWorkspace  VariableName=zz_SC_Pavail_sat  SaveFormat=Timeseries  SampleTime=1e-3
  zz_log_zz_SC_Vdc_den : ToWorkspace  VariableName=zz_SC_Vdc_den  SaveFormat=Timeseries  SampleTime=1e-3
  zz_log_zz_SC_Vguard : ToWorkspace  VariableName=zz_SC_Vguard  SaveFormat=Timeseries  SampleTime=1e-3
  Ibus_cmd : Outport
  Vsc_f_out : Outport  Port=2
  wires:
  Pmech/1 -> Pmech_f/1
  Pmech_f/1 -> P_avail/1, P_pos/1
  Pdead/1 -> P_avail/2, P_pos/2
  P_avail/1 -> P_avail_sat/1
  Vdc/1 -> Vdc_f/1
  Vdc_f/1 -> Vdc_den/1
  Vsc/1 -> Vsc_err/1
  Vsc_err/1 -> Vsc_gain/1
  Vsc_gain/1 -> Vsc_f/1
  Vsc_f/1 -> Vsc_err/2, V_margin/2, Vsc_f_out/1, V_lo_margin/1
  Vmax/1 -> V_margin/1
  V_margin/1 -> V_margin_gain/1
  V_margin_gain/1 -> V_guard/1
  P_avail_sat/1 -> P_abs/1, zz_log_zz_SC_Pavail_sat/1
  V_guard/1 -> P_abs/2, zz_log_zz_SC_Vguard/1
  Enable/1 -> P_abs/3, P_dis/3
  Vdc_den/1 -> I_abs/2, zz_log_zz_SC_Vdc_den/1
  I_abs/1 -> Sign/1
  Sign/1 -> Ibus_cmd/1
  P_pos/1 -> P_pos_sat/1
  P_pos_sat/1 -> Kdis/1
  Vmin/1 -> V_lo_margin/2
  V_lo_margin/1 -> V_lo_gain/1
  V_lo_gain/1 -> V_lo_guard/1
  Kdis/1 -> P_dis/1
  V_lo_guard/1 -> P_dis/2
  P_dis/1 -> P_net/1
  P_abs/1 -> P_net/2
  P_net/1 -> I_abs/1
